simulink model "Wind_Turbine_Flexible_Blades"  (R2025a)
settings: Solver=ode15s  StartTime=0.0  StopTime=10  RelTol=1e-5  EnableMultiTasking=on
PreLoadFcn:
  | load ss_cantilever_pva.mat
  | warning('off','Simulink:SL_SaveWithParameterizedLinks_Warning');
PostLoadFcn:
  | loadMass = 20; %kg
InitFcn:
  | cantilever1=cantilever_aluminum;
  | load1.mass = 20 ; %kg
  | load1.inertia = eye(3) ; % assume point mass
  | load2=load1;
  | load2.angle = 35 * pi / 180;
undefined symbols (not defined in the file or in its folder): Extr_Data_Ellipse, WT_Params, X, Y, Z
libraries: sm_lib x22, nesl_utility x7, Pitch_System_Lib x3, Hub_Axis_Lib x1
Description:
  | Copyright 2009-2025 The MathWorks, Inc. MathWorks, Inc.
settings Model: Creator=smiller  LastModifiedBy=smiller
settings SolverCC: AlgebraicLoopSolver=TrustRegion
settings DataIOCC: LimitDataPoints=on  SaveFormat=Array  SignalLoggingSaveFormat=ModelDataLogs  ReturnWorkspaceOutputs=off
settings OptimizationCC: ReuseModelBlockBuffer=off  ExpressionDepthLimit=2147483647.0  InitFltsAndDblsToZero=on  LifeSpan=inf
settings DebuggingCC: AlgebraicLoopMsg=none  ArtificialAlgebraicLoopMsg=none  UnderspecifiedInitializationDetection=Classic  MergeDetectMultiDrivingBlocksExec=none  FcnCallInpInsideContextMsg=warning  UnconnectedInputMsg=warning  UnconnectedOutputMsg=warning  UnconnectedLineMsg=warning  AllowSymbolicDim=off  StateNameClashWarn=warning  PregeneratedLibrarySubsystemCodeDiagnostic=none  SFUnexpectedBacktrackingDiag=warning  SFNoUnconditionalDefaultTransitionDiag=warning  SFExecutionAtInitializationDiag=none  ArithmeticOperatorsInVariantConditions=warning
settings HardwareCC: ProdBitPerPointer=32.0  ProdBitPerSizeT=32.0  ProdBitPerPtrDiffT=32.0  ProdLargestAtomicFloat=None  ProdIntDivRoundTo=Undefined  ProdEndianess=Unspecified  ProdWordSize=32.0  ProdHWDeviceType=32-bit Generic
settings ModelReferenceCC: EnableRefExpFcnMdlSchedulingChecks=on  PropagateSignalLabelsOutOfModel=off
settings SFSimCC: SimUseLocalCustomCode=off  CustomCodeUndefinedFunction=UseInterfaceOnly
settings RTWCC: RTWUseLocalCustomCode=off  GPUComputeCapability=3.5  DLArmComputeVersion=19.05
settings CodeAppCC: StateflowObjectComments=on
settings GRTTargetCC: TargetLangStandard=C89/C90 (ANSI)  CombineOutputUpdateFcns=off  GRTInterface=on
settings ConfigComp: CovMetricSettings=dw  CovSaveCumulativeToWorkspaceVar=on  CovSaveSingleToWorkspaceVar=on  CovExternalEMLEnable=off  CovSFcnEnable=off
settings SimscapeCC: SimscapeNormalizeSystem=off  SimscapeNominalValues="[{\"value\":\"10\",\"unit\":\"V\"},{\"value\":\"1\",\"unit\":\"A\"},{\"value\":\"10\",\"unit\":\"N*m\"},{\"value\":\"10\",\"unit\":\"bar\"},{\"value\":\"100\",\"unit\":\"kJ/kg\"},{\"value\":\"1\",\"unit\":\"kW\"},{\"value\":\"300\",\"unit\":\"K\"},{\"value\":\"100\",\"unit\":\"cm^3/s\"},{\"value\":\"1\",\"unit\":\"kN\"},{\"value\":\"1\",\"unit\":\"g/cm^3\"},{\"value\":\"1\",\"unit\":\"l\"},{\"value\":\"1\",\"unit\":\"cm^2\"},{\"value\":\"60\",\"unit\":\"Hz\"}]"
settings ConfigurationSet: Description=SimMechanics 2G
settings ExplorerConfigSet: InternalSimMechanicsExplorerSettings="<ExplorerConfiguration><canonicalview>default</canonicalview><AnimationSetting><BasePlaybackSpeed>1.0</BasePlaybackSpeed><PlaybackSpeedFactor>1.0</PlaybackSpeedFactor></AnimationSetting><TilePanel><TileInfo><Tiles Columns=\"1\" Count=\"1\" Rows=\"1\"><Column Weight=\"1\"/><Row Weight=\"1\"/><Tile Height=\"1\" Width=\"1\" X=\"0\" Y=\"0\"/></Tiles></TileInfo><SceneInfo><SceneViewer><BGColor><R>1</R><G>1</G><B>1</B></BGColor><Camera><DoPerspective>off</DoPerspective><Position><X>22.7951904532356409</X><Y>25.5078554918571712</Y><Z>43.6986236453718746</Z></Position><Center><X>-2.12432004859473977</X><Y>6.83325398558179486</Y><Z>-1.8734629381775747</Z></Center><Up><X>-0.455754206605199275</X><Y>0.882954249233147026</Y><Z>-0.112605048389475049</Z></Up><ViewLimDist>1</ViewLimDist><YLim>36.0998057556152361</YLim><XLim>37.6274144624230047</XLim></Camera></SceneViewer></SceneInfo></TilePanel><MechEditorPanel><Cameras/><GfxPanelCameraMap/><VideoCreator><PlaybackSpeedRatio>1.0</PlaybackSpeedRatio><FrameRate>30</FrameRate><VideoFormat>Motion JPEG AVI</VideoFormat><FrameSize>auto</FrameSize></VideoCreator></MechEditorPanel></ExplorerConfiguration>"

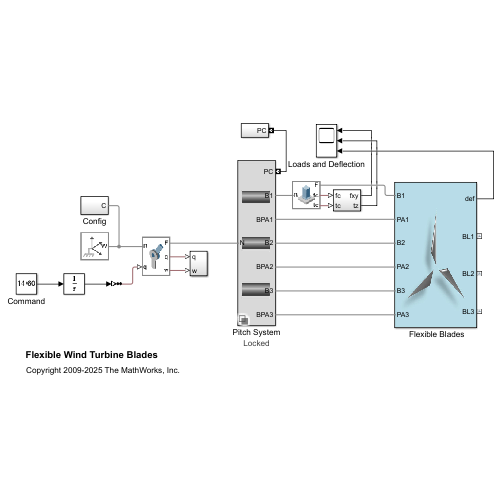
[thumbnail: Simulink's stored preview of the top-level diagram]
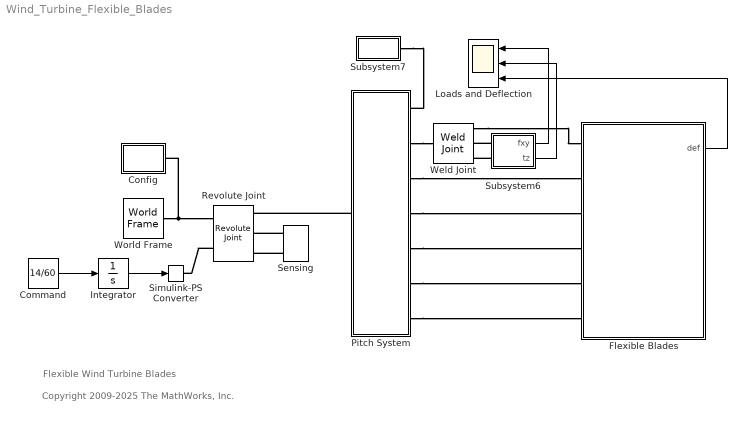
== system Wind_Turbine_Flexible_Blades ==
  note: Copyright 2009-2025 The MathWorks, Inc.
  note: Flexible Wind Turbine Blades
  " Flexible Blades" : Subsystem
      mask Display: image('Blades_IMAGE.jpg');
  Command : Constant  Value=14/60
  Config : Subsystem
  Integrator : Integrator
  Loads and Deflection : Scope  NumInputPorts=3
      settings: ActiveDisplayYMinimum=-4.81536855554E+6  ActiveDisplayYMaximum=1.42317027303E+6  DataLoggingVariableName=ScopeData3
  Pitch System : Subsystem  Tag=CustomStyle  Variant=on  VariantControlMode=label  LabelModeActiveChoice=Locked
      settings: AttributesFormatString=%<ActiveVariant>
      mask Display:
      | blk = wind_turbine_activeVariantBlock(gcb);
      | eval(get_param(blk, 'MaskDisplay'));
  Revolute Joint : sm_lib/Joints/Revolute Joint  JointMode=Normal  CompositeWrenchDir=FollowerOnBase  CompositeWrenchFrame=BaseFrame  SenseConstraintForce=off  SenseConstraintTorque=off  SenseTotalForce=off  SenseTotalTorque=off  PositionTargetSpecify=on  PositionTargetPriority=High  PositionTargetValue=0  PositionTargetValueUnits=deg  VelocityTargetSpecify=off  VelocityTargetPriority=High  VelocityTargetValue=0  VelocityTargetValueUnits=deg/s  EquilibriumPosition=0  EquilibriumPositionUnits=deg  SpringStiffness=0  SpringStiffnessUnits=N*m/deg  DampingCoefficient=0  DampingCoefficientUnits=N*m/(deg/s)  LowerLimitSpecify=off  LowerLimitBound=-90  LowerLimitBoundUnits=deg  LowerLimitStiffness=1e4  LowerLimitStiffnessUnits=N*m/deg  LowerLimitDamping=10  LowerLimitDampingUnits=N*m/(deg/s)  LowerLimitTransitionRegionWidth=0.1  LowerLimitTransitionRegionWidthUnits=deg  UpperLimitSpecify=off  UpperLimitBound=90  UpperLimitBoundUnits=deg  UpperLimitStiffness=1e4  UpperLimitStiffnessUnits=N*m/deg  UpperLimitDamping=10  UpperLimitDampingUnits=N*m/(deg/s)  UpperLimitTransitionRegionWidth=0.1  UpperLimitTransitionRegionWidthUnits=deg  TorqueActuationMode=ComputedTorque  MotionActuationMode=InputMotion  SensePosition=on  SenseVelocity=on  SenseAcceleration=off  SenseTorqueForce=off  SenseLowerLimitTorqueForce=off  SenseUpperLimitTorqueForce=off
  Sensing : Hub_Axis_Lib/Rotate/Sensing  SystemSampleTime=-1  VariantActivationTime=update diagram  EmptyChoice=off  PassThrough=off  PassThroughVariantControl=(default)  EmptyChoiceVariantControl=(default)  AllowFlexibleInterface=on  Latency=0  AutoFrameSizeCalculation=off
  Simulink-PS Converter : nesl_utility/Simulink-PS Converter  PhysicalDomain=network_engine_domain  SubClassName=ps_input  LeftPortType=input  RightPortType=output  PseudoPeriodic=off  Frequencies=[]  NoiseDistribution=none  NoiseParameters=[]  Unit=rev  AffineConversion=off  FilteringAndDerivatives=filter  SimscapeFilterOrder=2  InputFilterTimeConstant=4  UdotUserProvided=0
  Subsystem6 : Subsystem
  Subsystem7 : Subsystem
  Weld Joint : sm_lib/Joints/Weld Joint  JointMode=Normal  CompositeWrenchDir=FollowerOnBase  CompositeWrenchFrame=BaseFrame  SenseConstraintForce=on  SenseConstraintTorque=on  SenseTotalForce=off  SenseTotalTorque=off
  World Frame : sm_lib/Frames and Transforms/World Frame
  wires:
  Command/1 -> Integrator/1
  Subsystem6/1(fxy) -> Loads and Deflection/1
  Subsystem6/2(tz) -> Loads and Deflection/2
  Integrator/1 -> Simulink-PS Converter/1
  " Flexible Blades"/1(def) -> Loads and Deflection/3
  connections:
  Pitch System/LConn6 -- " Flexible Blades"/LConn5
  Pitch System/LConn5 -- " Flexible Blades"/LConn4
  Pitch System/RConn1 -- Revolute Joint/RConn1
  Sensing/LConn1 -- Revolute Joint/RConn2
  Pitch System/LConn2 -- Weld Joint/LConn1
  Pitch System/LConn4 -- " Flexible Blades"/LConn3
  Pitch System/LConn3 -- " Flexible Blades"/LConn2
  Sensing/LConn2 -- Revolute Joint/RConn3
  Pitch System/LConn7 -- " Flexible Blades"/LConn6
  World Frame/RConn1 -- Config/LConn1 -- Revolute Joint/LConn1
  Weld Joint/RConn1 -- " Flexible Blades"/LConn1
  Subsystem6/LConn1 -- Weld Joint/RConn2
  Subsystem6/LConn2 -- Weld Joint/RConn3
  Revolute Joint/LConn2 -- Simulink-PS Converter/RConn1
  Subsystem7/LConn1 -- Pitch System/LConn1

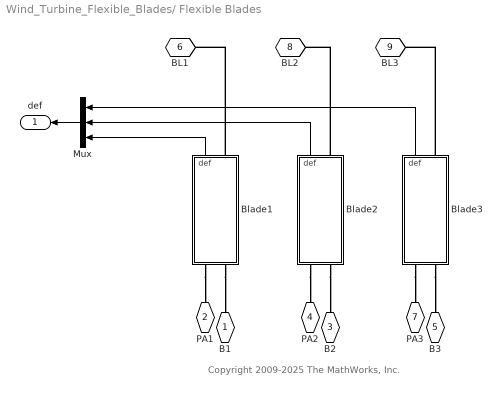
== system Wind_Turbine_Flexible_Blades/ Flexible Blades ==
  note: Copyright 2009-2025 The MathWorks, Inc.
  Blade1 : Subsystem
  Blade2 : Subsystem
  Blade3 : Subsystem
  Mux : Mux  Inputs=3
  B1 : PMIOPort  Tag=PMCPort  Side=Left
  PA1 : PMIOPort  Tag=PMCPort  Port=2  Side=Left
  B2 : PMIOPort  Tag=PMCPort  Port=3  Side=Left
  PA2 : PMIOPort  Tag=PMCPort  Port=4  Side=Left
  B3 : PMIOPort  Tag=PMCPort  Port=5  Side=Left
  BL1 : PMIOPort  Tag=PMCPort  Port=6  Side=Right
  PA3 : PMIOPort  Tag=PMCPort  Port=7  Side=Left
  BL2 : PMIOPort  Tag=PMCPort  Port=8  Side=Right
  BL3 : PMIOPort  Tag=PMCPort  Port=9  Side=Right
  def : Outport  VectorParamsAs1DForOutWhenUnconnected=off
  wires:
  Blade1/1(def) -> Mux/3
  Blade2/1(def) -> Mux/2
  Blade3/1(def) -> Mux/1
  Mux/1 -> def/1
  connections:
  Blade3/LConn1 -- PA3/RConn1
  Blade3/RConn1 -- BL3/RConn1
  Blade3/LConn2 -- B3/RConn1
  Blade2/LConn2 -- B2/RConn1
  Blade2/RConn1 -- BL2/RConn1
  Blade2/LConn1 -- PA2/RConn1
  Blade1/LConn2 -- B1/RConn1
  Blade1/LConn1 -- PA1/RConn1
  Blade1/RConn1 -- BL1/RConn1

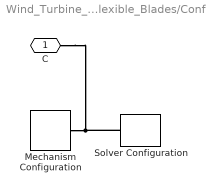
== system Wind_Turbine_Flexible_Blades/Config ==
  Mechanism Configuration : sm_lib/Utilities/Mechanism Configuration  UniformGravity=Constant  GravityVector=[0 0 -9.81]  GravityVectorUnits=m/s^2  LinearizationDelta=0.001  JointModeTransitionNonlinearIterations=2
  Solver Configuration : nesl_utility/Solver Configuration  PhysicalDomain=network_engine_domain  SubClassName=solver  LeftPortType=input  RightPortType=generic  Tones=[]  Harmonics=[]  SimulateNoise=off  Profile=off  UseLocalSampling=off  EnableSwitchedLinearOptims=on  FrequencyDomain=off  UseCCode=off  RelTol=0.001  AbsTol=1e-06  MinStep=1e-09  ToWorkspace=off  RevertToSquareIcSolve=off  NumHomotopyIterations=100  PhasorMode=off  PhasorModeNumHarmonics=1  ConsistencySolver=NEWTON_FTOL  IndexReductionMethod=DerivativeReplacement  DoDC=off  ResidualTolerance=1e-9  ConsistencyTolSource=GLOBAL  ConsistencyAbsTol=0.001  ConsistencyRelTol=0.001  ConsistencyTolFactor=0.001  UseLocalSolver=off  LocalSolverChoice=NE_BACKWARD_EULER_ADVANCER  ResolveIndetEquations=on  FunctionEvalNumThread=1  LocalSolverSampleTime=.001  DoFixedCost=off  MaxNonlinIter=3  MaxModeIter=2  ComputeImpulses=off  ImpulseIterations=2  LinearAlgebra=Sparse  LinearAlgebraNumThread=0  EquationFormulation=NE_TIME_EF  DelaysMemoryBudget=1024  AutomaticFiltering=on  FilteringTimeConstant=0.001  PartitionStorageMethod=AS_NEEDED  PartitionMemoryBudget=1024  PartitionMethod=FAST  MultibodyUseLocalSolver=off  MultibodyLocalSolverChoice=ODE1  MultibodyLocalSolverSampleTime=0.001
  C : PMIOPort  Side=Left
  connections:
  Solver Configuration/RConn1 -- C/RConn1 -- Mechanism Configuration/RConn1

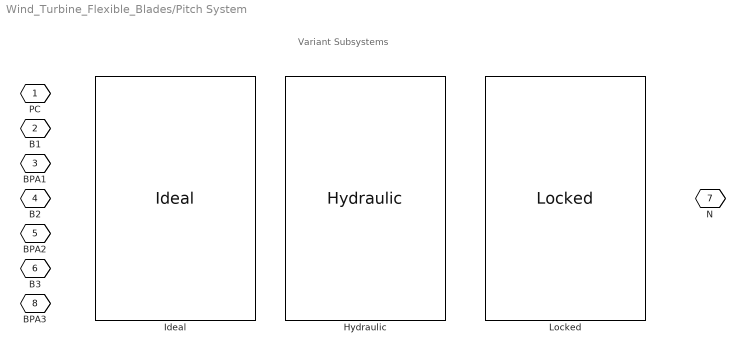
== system Wind_Turbine_Flexible_Blades/Pitch System ==
  note: Variant Subsystems
  Hydraulic : Pitch_System_Lib/Hydraulic  SystemSampleTime=-1  VariantControl=Hydraulic  VariantActivationTime=update diagram  EmptyChoice=off  PassThrough=off  PassThroughVariantControl=(default)  EmptyChoiceVariantControl=(default)  AllowFlexibleInterface=on  Latency=0  AutoFrameSizeCalculation=off
  Ideal : Pitch_System_Lib/Ideal  SystemSampleTime=-1  VariantControl=Ideal  VariantActivationTime=update diagram  EmptyChoice=off  PassThrough=off  PassThroughVariantControl=(default)  EmptyChoiceVariantControl=(default)  AllowFlexibleInterface=on  Latency=0  AutoFrameSizeCalculation=off
  Locked : Pitch_System_Lib/Locked  SystemSampleTime=-1  VariantControl=Locked  VariantActivationTime=update diagram  EmptyChoice=off  PassThrough=off  PassThroughVariantControl=(default)  EmptyChoiceVariantControl=(default)  AllowFlexibleInterface=on  Latency=0  AutoFrameSizeCalculation=off
  PC : PMIOPort  Tag=PMCPort  Side=Left
  B1 : PMIOPort  Tag=PMCPort  Port=2  Side=Left
  BPA1 : PMIOPort  Tag=PMCPort  Port=3  Side=Left
  B2 : PMIOPort  Tag=PMCPort  Port=4  Side=Left
  BPA2 : PMIOPort  Tag=PMCPort  Port=5  Side=Left
  B3 : PMIOPort  Tag=PMCPort  Port=6  Side=Left
  N : PMIOPort  Tag=PMCPort  Port=7  Side=Right
  BPA3 : PMIOPort  Tag=PMCPort  Port=8  Side=Left

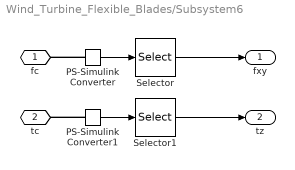
== system Wind_Turbine_Flexible_Blades/Subsystem6 ==
  PS-Simulink Converter : nesl_utility/PS-Simulink Converter  PhysicalDomain=network_engine_domain  SubClassName=ps_output  LeftPortType=input  RightPortType=output  PseudoPeriodic=off  Frequencies=[]  VectorFormat=1-D array  Unit=1  AffineConversion=off
  PS-Simulink Converter1 : nesl_utility/PS-Simulink Converter  PhysicalDomain=network_engine_domain  SubClassName=ps_output  LeftPortType=input  RightPortType=output  PseudoPeriodic=off  Frequencies=[]  VectorFormat=1-D array  Unit=1  AffineConversion=off
  Selector : Selector  InputPortWidth=3  IndexOptions=Index vector (dialog)  Indices=[1 2]  OutputSizes=1
  Selector1 : Selector  InputPortWidth=3  IndexOptions=Index vector (dialog)  Indices=[3]  OutputSizes=1
  fc : PMIOPort  Side=Left
  tc : PMIOPort  Port=2  Side=Left
  fxy : Outport  VectorParamsAs1DForOutWhenUnconnected=off
  tz : Outport  Port=2  VectorParamsAs1DForOutWhenUnconnected=off
  wires:
  PS-Simulink Converter/1 -> Selector/1
  PS-Simulink Converter1/1 -> Selector1/1
  Selector/1 -> fxy/1
  Selector1/1 -> tz/1
  connections:
  PS-Simulink Converter1/LConn1 -- tc/RConn1
  PS-Simulink Converter/LConn1 -- fc/RConn1

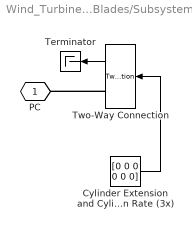
== system Wind_Turbine_Flexible_Blades/Subsystem7 ==
  Cylinder Extension and Cylinder Extension Rate (3x) : Constant  Value=[0 0 0 0 0 0]
  Terminator : Terminator
  Two-Way Connection : TwoWayConnection
  PC : PMIOPort  Tag=PMCPort  Side=Left
  wires:
  Two-Way Connection/1 -> Terminator/1
  Cylinder Extension and Cylinder Extension Rate (3x)/1 -> Two-Way Connection/1
  connections:
  Two-Way Connection/RConn1 -- PC/RConn1

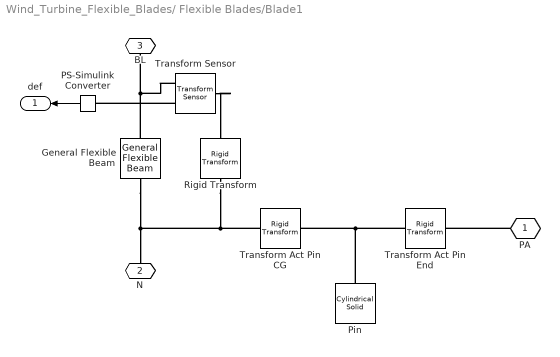
== system Wind_Turbine_Flexible_Blades/ Flexible Blades/Blade1 ==
  General Flexible Beam : sm_lib/Body Elements/Flexible Bodies/Beams/General Flexible Beam  ExtrusionCrossSection=Extr_Data_Ellipse(0.5,1.5,0,359,1)  ExtrusionCrossSectionUnits=m  ExtrusionLength=40  ExtrusionLengthUnits=m  StiffnessAndInertiaType=CalculateFromGeometry  Density=2700  DensityUnits=kg/m^3  ModuliType=YoungsPoissons  YoungsModulus=70  YoungsModulusUnits=GPa  PoissonsRatio=0.33  ShearModulus=26  ShearModulusUnits=GPa  GeometricCentroid=[0 0]  GeometricCentroidUnits=m  BendingCentroid=[0 0]  BendingCentroidUnits=m  ShearCenter=[0 0]  ShearCenterUnits=m  AxialRigidity=1  AxialRigidityUnits=Pa*m^2  FlexuralRigidity=[1 1]  FlexuralRigidityUnits=Pa*m^4  CrossFlexuralRigidity=0  CrossFlexuralRigidityUnits=Pa*m^4  TorsionalRigidity=1  TorsionalRigidityUnits=Pa*m^4  CenterOfMass=[0 0]  CenterOfMassUnits=m  MassPerUnitLength=1  MassPerUnitLengthUnits=kg/m  MassMomentOfInertiaDensity=[1 1]  MassMomentOfInertiaDensityUnits=kg*m  MassProductOfInertiaDensity=0  MassProductOfInertiaDensityUnits=kg*m  DampingType=Proportional  ProportionalDampingAlpha=0  ProportionalDampingAlphaUnits=1/s  ProportionalDampingBeta=0.001  ProportionalDampingBetaUnits=s  UniformModalDampingRatio=0.01  NumElements=1  ReferenceConditionsType=LinearizedMeanAxes  DoExposeReferenceFrame=off  ReductionType=None  NumRetainedModes=1  GraphicType=FromGeometry  GraphicVisPropType=SimpleVisualProperties  GraphicDiffuseColor=[0.5 0.5 0.5]  GraphicOpacity=1.0  GraphicSpecularColor=[0.5 0.5 0.5 1.0]  GraphicAmbientColor=[0.15 0.15 0.15 1.0]  GraphicEmissiveColor=[0.0 0.0 0.0 1.0]  GraphicShininess=75  DoExposeZminFrame=on  DoExposeZmaxFrame=on  SerializedFrames=<Frames/>
  PS-Simulink Converter : nesl_utility/PS-Simulink Converter  PhysicalDomain=network_engine_domain  SubClassName=ps_output  LeftPortType=input  RightPortType=output  PseudoPeriodic=off  Frequencies=[]  VectorFormat=1-D array  Unit=1  AffineConversion=off
  Pin : sm_lib/Body Elements/Cylindrical Solid  CylinderRadius=0.1  CylinderRadiusUnits=m  CylinderLength=-WT_Params.Blade.Actuator_Offset.y  CylinderLengthUnits=m  ExportEntireGeometry=off  InertiaType=PointMass  BasedOnType=Density  Density=1000  DensityUnits=kg/(m^3)  Mass=0.001  MassUnits=kg  CenterOfMass=[0 0 0]  CenterOfMassUnits=m  MomentsOfInertia=[1 1 1]  MomentsOfInertiaUnits=kg*m^2  ProductsOfInertia=[0 0 0]  ProductsOfInertiaUnits=kg*m^2  GraphicType=FromGeometry  MarkerShape=Sphere  MarkerSize=10  GraphicVisPropType=SimpleVisualProperties  GraphicDiffuseColor=[0.6 0.2 0.0]  GraphicOpacity=1.0  GraphicSpecularColor=[0.5 0.5 0.5 1.0]  GraphicAmbientColor=[0.15 0.15 0.15 1.0]  GraphicEmissiveColor=[0.0 0.0 0.0 1.0]  GraphicShininess=75  DoExposeReferenceFrame=on  SerializedFrames=<Frames/>
  Rigid Transform : sm_lib/Frames and Transforms/Rigid Transform  RotationMethod=None  FollAlignAxisA=+X  BaseAlignAxisA=+Y  FollAlignAxisB=+Y  BaseAlignAxisB=+Z  RotationStandardAxis=+Z  RotationAngle=0.0  RotationAngleUnits=deg  RotationArbitraryAxis=[0 0 1]  RotationSequenceAxes=FollowerAxes  RotationSequence=XYX  RotationSequenceAngles=[0 0 0]  RotationSequenceAnglesUnits=deg  RotationMatrix=[1 0 0; 0 1 0; 0 0 1]  Quaternion=[1 0 0 0]  TranslationMethod=StandardAxis  TranslationCartesianOffset=[0 0 0]  TranslationCartesianOffsetUnits=m  TranslationStandardAxis=+Z  TranslationStandardOffset=40  TranslationStandardOffsetUnits=m  TranslationROffset=0  TranslationROffsetUnits=m  TranslationThetaOffset=0  TranslationThetaOffsetUnits=deg  TranslationZOffset=0  TranslationZOffsetUnits=m
  Transform Act Pin CG : sm_lib/Frames and Transforms/Rigid Transform  RotationMethod=None  FollAlignAxisA=+X  BaseAlignAxisA=+Y  FollAlignAxisB=+Y  BaseAlignAxisB=+Z  RotationStandardAxis=+Z  RotationAngle=0  RotationAngleUnits=deg  RotationArbitraryAxis=[0 0 1]  RotationSequenceAxes=FollowerAxes  RotationSequence=XYX  RotationSequenceAngles=[0 0 0]  RotationSequenceAnglesUnits=deg  RotationMatrix=[1 0 0; 0 1 0; 0 0 1]  Quaternion=[1 0 0 0]  TranslationMethod=Cartesian  TranslationCartesianOffset=[0 WT_Params.Blade.Actuator_Offset.z WT_Params.Blade.Actuator_Offset.y/2]  TranslationCartesianOffsetUnits=m  TranslationStandardAxis=+Z  TranslationStandardOffset=0  TranslationStandardOffsetUnits=m  TranslationROffset=0  TranslationROffsetUnits=m  TranslationThetaOffset=0  TranslationThetaOffsetUnits=deg  TranslationZOffset=0  TranslationZOffsetUnits=m
  Transform Act Pin End : sm_lib/Frames and Transforms/Rigid Transform  RotationMethod=None  FollAlignAxisA=+X  BaseAlignAxisA=+Y  FollAlignAxisB=+Y  BaseAlignAxisB=+Z  RotationStandardAxis=+Z  RotationAngle=0  RotationAngleUnits=deg  RotationArbitraryAxis=[0 0 1]  RotationSequenceAxes=FollowerAxes  RotationSequence=XYX  RotationSequenceAngles=[0 0 0]  RotationSequenceAnglesUnits=deg  RotationMatrix=[1 0 0; 0 1 0; 0 0 1]  Quaternion=[1 0 0 0]  TranslationMethod=Cartesian  TranslationCartesianOffset=[0 0 WT_Params.Blade.Actuator_Offset.y/2]  TranslationCartesianOffsetUnits=m  TranslationStandardAxis=+Z  TranslationStandardOffset=0  TranslationStandardOffsetUnits=m  TranslationROffset=0  TranslationROffsetUnits=m  TranslationThetaOffset=0  TranslationThetaOffsetUnits=deg  TranslationZOffset=0  TranslationZOffsetUnits=m
  Transform Sensor : sm_lib/Frames and Transforms/Transform Sensor  MeasurementFrame=World  RotationSequence=XYX  SenseAngle=off  SenseAxis=off  SenseQ=off  SenseR=off  SenseRotationSequence=off  SenseOmegaX=off  SenseOmegaY=off  SenseOmegaZ=off  SenseOmega=off  SenseQDot=off  SenseRDot=off  SenseRotationSequenceDot=off  SenseAlphaX=off  SenseAlphaY=off  SenseAlphaZ=off  SenseAlpha=off  SenseQDDot=off  SenseRDDot=off  SenseX=off  SenseY=off  SenseZ=off  SenseXYZ=off  SenseRad=on  SenseAzim=off  SenseDist=off  SenseInc=off  SenseXDot=off  SenseYDot=off  SenseZDot=off  SenseXYZDot=off  SenseRadDot=off  SenseAzimDot=off  SenseDistDot=off  SenseIncDot=off  SenseXDDot=off  SenseYDDot=off  SenseZDDot=off  SenseXYZDDot=off  SenseRadDDot=off  SenseAzimDDot=off  SenseDistDDot=off  SenseIncDDot=off
  PA : PMIOPort  Side=Left
  N : PMIOPort  Port=2  Side=Left
  BL : PMIOPort  Port=3  Side=Right
  def : Outport  VectorParamsAs1DForOutWhenUnconnected=off
  wires:
  PS-Simulink Converter/1 -> def/1
  connections:
  Pin/RConn1 -- Transform Act Pin End/LConn1 -- Transform Act Pin CG/RConn1
  PA/RConn1 -- Transform Act Pin End/RConn1
  General Flexible Beam/RConn1 -- Transform Sensor/RConn1 -- BL/RConn1
  Transform Act Pin CG/LConn1 -- Rigid Transform/LConn1 -- General Flexible Beam/LConn1 -- N/RConn1
  Transform Sensor/LConn1 -- Rigid Transform/RConn1
  Transform Sensor/RConn2 -- PS-Simulink Converter/LConn1

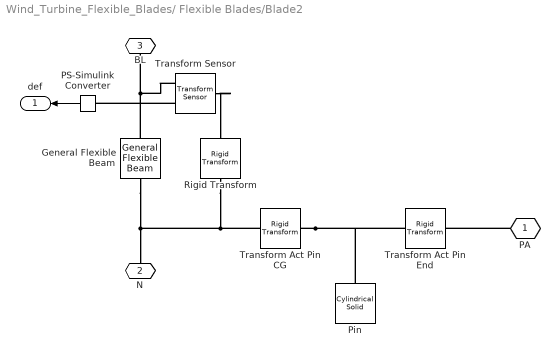
== system Wind_Turbine_Flexible_Blades/ Flexible Blades/Blade2 ==
  General Flexible Beam : sm_lib/Body Elements/Flexible Bodies/Beams/General Flexible Beam  ExtrusionCrossSection=Extr_Data_Ellipse(0.5,1.5,0,359,1)  ExtrusionCrossSectionUnits=m  ExtrusionLength=40  ExtrusionLengthUnits=m  StiffnessAndInertiaType=CalculateFromGeometry  Density=2700  DensityUnits=kg/m^3  ModuliType=YoungsPoissons  YoungsModulus=70  YoungsModulusUnits=GPa  PoissonsRatio=0.33  ShearModulus=26  ShearModulusUnits=GPa  GeometricCentroid=[0 0]  GeometricCentroidUnits=m  BendingCentroid=[0 0]  BendingCentroidUnits=m  ShearCenter=[0 0]  ShearCenterUnits=m  AxialRigidity=1  AxialRigidityUnits=Pa*m^2  FlexuralRigidity=[1 1]  FlexuralRigidityUnits=Pa*m^4  CrossFlexuralRigidity=0  CrossFlexuralRigidityUnits=Pa*m^4  TorsionalRigidity=1  TorsionalRigidityUnits=Pa*m^4  CenterOfMass=[0 0]  CenterOfMassUnits=m  MassPerUnitLength=1  MassPerUnitLengthUnits=kg/m  MassMomentOfInertiaDensity=[1 1]  MassMomentOfInertiaDensityUnits=kg*m  MassProductOfInertiaDensity=0  MassProductOfInertiaDensityUnits=kg*m  DampingType=Proportional  ProportionalDampingAlpha=0  ProportionalDampingAlphaUnits=1/s  ProportionalDampingBeta=0.001  ProportionalDampingBetaUnits=s  UniformModalDampingRatio=0.01  NumElements=1  ReferenceConditionsType=LinearizedMeanAxes  DoExposeReferenceFrame=off  ReductionType=None  NumRetainedModes=1  GraphicType=FromGeometry  GraphicVisPropType=SimpleVisualProperties  GraphicDiffuseColor=[0.5 0.5 0.5]  GraphicOpacity=1.0  GraphicSpecularColor=[0.5 0.5 0.5 1.0]  GraphicAmbientColor=[0.15 0.15 0.15 1.0]  GraphicEmissiveColor=[0.0 0.0 0.0 1.0]  GraphicShininess=75  DoExposeZminFrame=on  DoExposeZmaxFrame=on  SerializedFrames=<Frames/>
  PS-Simulink Converter : nesl_utility/PS-Simulink Converter  PhysicalDomain=network_engine_domain  SubClassName=ps_output  LeftPortType=input  RightPortType=output  PseudoPeriodic=off  Frequencies=[]  VectorFormat=1-D array  Unit=1  AffineConversion=off
  Pin : sm_lib/Body Elements/Cylindrical Solid  CylinderRadius=0.1  CylinderRadiusUnits=m  CylinderLength=-WT_Params.Blade.Actuator_Offset.y  CylinderLengthUnits=m  ExportEntireGeometry=off  InertiaType=PointMass  BasedOnType=Density  Density=1000  DensityUnits=kg/(m^3)  Mass=0.001  MassUnits=kg  CenterOfMass=[0 0 0]  CenterOfMassUnits=m  MomentsOfInertia=[1 1 1]  MomentsOfInertiaUnits=kg*m^2  ProductsOfInertia=[0 0 0]  ProductsOfInertiaUnits=kg*m^2  GraphicType=FromGeometry  MarkerShape=Sphere  MarkerSize=10  GraphicVisPropType=SimpleVisualProperties  GraphicDiffuseColor=[0.6 0.2 0.0]  GraphicOpacity=1.0  GraphicSpecularColor=[0.5 0.5 0.5 1.0]  GraphicAmbientColor=[0.15 0.15 0.15 1.0]  GraphicEmissiveColor=[0.0 0.0 0.0 1.0]  GraphicShininess=75  DoExposeReferenceFrame=on  SerializedFrames=<Frames/>
  Rigid Transform : sm_lib/Frames and Transforms/Rigid Transform  RotationMethod=None  FollAlignAxisA=+X  BaseAlignAxisA=+Y  FollAlignAxisB=+Y  BaseAlignAxisB=+Z  RotationStandardAxis=+Z  RotationAngle=0.0  RotationAngleUnits=deg  RotationArbitraryAxis=[0 0 1]  RotationSequenceAxes=FollowerAxes  RotationSequence=XYX  RotationSequenceAngles=[0 0 0]  RotationSequenceAnglesUnits=deg  RotationMatrix=[1 0 0; 0 1 0; 0 0 1]  Quaternion=[1 0 0 0]  TranslationMethod=StandardAxis  TranslationCartesianOffset=[0 0 0]  TranslationCartesianOffsetUnits=m  TranslationStandardAxis=+Z  TranslationStandardOffset=40  TranslationStandardOffsetUnits=m  TranslationROffset=0  TranslationROffsetUnits=m  TranslationThetaOffset=0  TranslationThetaOffsetUnits=deg  TranslationZOffset=0  TranslationZOffsetUnits=m
  Transform Act Pin CG : sm_lib/Frames and Transforms/Rigid Transform  RotationMethod=None  FollAlignAxisA=+X  BaseAlignAxisA=+Y  FollAlignAxisB=+Y  BaseAlignAxisB=+Z  RotationStandardAxis=+Z  RotationAngle=0  RotationAngleUnits=deg  RotationArbitraryAxis=[0 0 1]  RotationSequenceAxes=FollowerAxes  RotationSequence=XYX  RotationSequenceAngles=[0 0 0]  RotationSequenceAnglesUnits=deg  RotationMatrix=[1 0 0; 0 1 0; 0 0 1]  Quaternion=[1 0 0 0]  TranslationMethod=Cartesian  TranslationCartesianOffset=[0 WT_Params.Blade.Actuator_Offset.z WT_Params.Blade.Actuator_Offset.y/2]  TranslationCartesianOffsetUnits=m  TranslationStandardAxis=+Z  TranslationStandardOffset=0  TranslationStandardOffsetUnits=m  TranslationROffset=0  TranslationROffsetUnits=m  TranslationThetaOffset=0  TranslationThetaOffsetUnits=deg  TranslationZOffset=0  TranslationZOffsetUnits=m
  Transform Act Pin End : sm_lib/Frames and Transforms/Rigid Transform  RotationMethod=None  FollAlignAxisA=+X  BaseAlignAxisA=+Y  FollAlignAxisB=+Y  BaseAlignAxisB=+Z  RotationStandardAxis=+Z  RotationAngle=0  RotationAngleUnits=deg  RotationArbitraryAxis=[0 0 1]  RotationSequenceAxes=FollowerAxes  RotationSequence=XYX  RotationSequenceAngles=[0 0 0]  RotationSequenceAnglesUnits=deg  RotationMatrix=[1 0 0; 0 1 0; 0 0 1]  Quaternion=[1 0 0 0]  TranslationMethod=Cartesian  TranslationCartesianOffset=[0 0 WT_Params.Blade.Actuator_Offset.y/2]  TranslationCartesianOffsetUnits=m  TranslationStandardAxis=+Z  TranslationStandardOffset=0  TranslationStandardOffsetUnits=m  TranslationROffset=0  TranslationROffsetUnits=m  TranslationThetaOffset=0  TranslationThetaOffsetUnits=deg  TranslationZOffset=0  TranslationZOffsetUnits=m
  Transform Sensor : sm_lib/Frames and Transforms/Transform Sensor  MeasurementFrame=World  RotationSequence=XYX  SenseAngle=off  SenseAxis=off  SenseQ=off  SenseR=off  SenseRotationSequence=off  SenseOmegaX=off  SenseOmegaY=off  SenseOmegaZ=off  SenseOmega=off  SenseQDot=off  SenseRDot=off  SenseRotationSequenceDot=off  SenseAlphaX=off  SenseAlphaY=off  SenseAlphaZ=off  SenseAlpha=off  SenseQDDot=off  SenseRDDot=off  SenseX=off  SenseY=off  SenseZ=off  SenseXYZ=off  SenseRad=on  SenseAzim=off  SenseDist=off  SenseInc=off  SenseXDot=off  SenseYDot=off  SenseZDot=off  SenseXYZDot=off  SenseRadDot=off  SenseAzimDot=off  SenseDistDot=off  SenseIncDot=off  SenseXDDot=off  SenseYDDot=off  SenseZDDot=off  SenseXYZDDot=off  SenseRadDDot=off  SenseAzimDDot=off  SenseDistDDot=off  SenseIncDDot=off
  PA : PMIOPort  Side=Left
  N : PMIOPort  Port=2  Side=Left
  BL : PMIOPort  Port=3  Side=Right
  def : Outport  VectorParamsAs1DForOutWhenUnconnected=off
  wires:
  PS-Simulink Converter/1 -> def/1
  connections:
  Transform Sensor/RConn2 -- PS-Simulink Converter/LConn1
  Transform Sensor/LConn1 -- Rigid Transform/RConn1
  Rigid Transform/LConn1 -- Transform Act Pin CG/LConn1 -- N/RConn1 -- General Flexible Beam/LConn1
  Transform Sensor/RConn1 -- General Flexible Beam/RConn1 -- BL/RConn1
  PA/RConn1 -- Transform Act Pin End/RConn1
  Transform Act Pin CG/RConn1 -- Transform Act Pin End/LConn1 -- Pin/RConn1

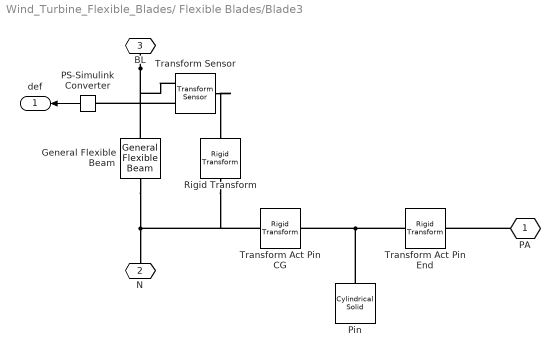
== system Wind_Turbine_Flexible_Blades/ Flexible Blades/Blade3 ==
  General Flexible Beam : sm_lib/Body Elements/Flexible Bodies/Beams/General Flexible Beam  ExtrusionCrossSection=Extr_Data_Ellipse(0.5,1.5,0,359,1)  ExtrusionCrossSectionUnits=m  ExtrusionLength=40  ExtrusionLengthUnits=m  StiffnessAndInertiaType=CalculateFromGeometry  Density=2700  DensityUnits=kg/m^3  ModuliType=YoungsPoissons  YoungsModulus=70  YoungsModulusUnits=GPa  PoissonsRatio=0.33  ShearModulus=26  ShearModulusUnits=GPa  GeometricCentroid=[0 0]  GeometricCentroidUnits=m  BendingCentroid=[0 0]  BendingCentroidUnits=m  ShearCenter=[0 0]  ShearCenterUnits=m  AxialRigidity=1  AxialRigidityUnits=Pa*m^2  FlexuralRigidity=[1 1]  FlexuralRigidityUnits=Pa*m^4  CrossFlexuralRigidity=0  CrossFlexuralRigidityUnits=Pa*m^4  TorsionalRigidity=1  TorsionalRigidityUnits=Pa*m^4  CenterOfMass=[0 0]  CenterOfMassUnits=m  MassPerUnitLength=1  MassPerUnitLengthUnits=kg/m  MassMomentOfInertiaDensity=[1 1]  MassMomentOfInertiaDensityUnits=kg*m  MassProductOfInertiaDensity=0  MassProductOfInertiaDensityUnits=kg*m  DampingType=Proportional  ProportionalDampingAlpha=0  ProportionalDampingAlphaUnits=1/s  ProportionalDampingBeta=0.001  ProportionalDampingBetaUnits=s  UniformModalDampingRatio=0.01  NumElements=1  ReferenceConditionsType=LinearizedMeanAxes  DoExposeReferenceFrame=off  ReductionType=None  NumRetainedModes=1  GraphicType=FromGeometry  GraphicVisPropType=SimpleVisualProperties  GraphicDiffuseColor=[0.5 0.5 0.5]  GraphicOpacity=1.0  GraphicSpecularColor=[0.5 0.5 0.5 1.0]  GraphicAmbientColor=[0.15 0.15 0.15 1.0]  GraphicEmissiveColor=[0.0 0.0 0.0 1.0]  GraphicShininess=75  DoExposeZminFrame=on  DoExposeZmaxFrame=on  SerializedFrames=<Frames/>
  PS-Simulink Converter : nesl_utility/PS-Simulink Converter  PhysicalDomain=network_engine_domain  SubClassName=ps_output  LeftPortType=input  RightPortType=output  PseudoPeriodic=off  Frequencies=[]  VectorFormat=1-D array  Unit=1  AffineConversion=off
  Pin : sm_lib/Body Elements/Cylindrical Solid  CylinderRadius=0.1  CylinderRadiusUnits=m  CylinderLength=-WT_Params.Blade.Actuator_Offset.y  CylinderLengthUnits=m  ExportEntireGeometry=off  InertiaType=PointMass  BasedOnType=Density  Density=1000  DensityUnits=kg/(m^3)  Mass=0.001  MassUnits=kg  CenterOfMass=[0 0 0]  CenterOfMassUnits=m  MomentsOfInertia=[1 1 1]  MomentsOfInertiaUnits=kg*m^2  ProductsOfInertia=[0 0 0]  ProductsOfInertiaUnits=kg*m^2  GraphicType=FromGeometry  MarkerShape=Sphere  MarkerSize=10  GraphicVisPropType=SimpleVisualProperties  GraphicDiffuseColor=[0.6 0.2 0.0]  GraphicOpacity=1.0  GraphicSpecularColor=[0.5 0.5 0.5 1.0]  GraphicAmbientColor=[0.15 0.15 0.15 1.0]  GraphicEmissiveColor=[0.0 0.0 0.0 1.0]  GraphicShininess=75  DoExposeReferenceFrame=on  SerializedFrames=<Frames/>
  Rigid Transform : sm_lib/Frames and Transforms/Rigid Transform  RotationMethod=None  FollAlignAxisA=+X  BaseAlignAxisA=+Y  FollAlignAxisB=+Y  BaseAlignAxisB=+Z  RotationStandardAxis=+Z  RotationAngle=0.0  RotationAngleUnits=deg  RotationArbitraryAxis=[0 0 1]  RotationSequenceAxes=FollowerAxes  RotationSequence=XYX  RotationSequenceAngles=[0 0 0]  RotationSequenceAnglesUnits=deg  RotationMatrix=[1 0 0; 0 1 0; 0 0 1]  Quaternion=[1 0 0 0]  TranslationMethod=StandardAxis  TranslationCartesianOffset=[0 0 0]  TranslationCartesianOffsetUnits=m  TranslationStandardAxis=+Z  TranslationStandardOffset=40  TranslationStandardOffsetUnits=m  TranslationROffset=0  TranslationROffsetUnits=m  TranslationThetaOffset=0  TranslationThetaOffsetUnits=deg  TranslationZOffset=0  TranslationZOffsetUnits=m
  Transform Act Pin CG : sm_lib/Frames and Transforms/Rigid Transform  RotationMethod=None  FollAlignAxisA=+X  BaseAlignAxisA=+Y  FollAlignAxisB=+Y  BaseAlignAxisB=+Z  RotationStandardAxis=+Z  RotationAngle=0  RotationAngleUnits=deg  RotationArbitraryAxis=[0 0 1]  RotationSequenceAxes=FollowerAxes  RotationSequence=XYX  RotationSequenceAngles=[0 0 0]  RotationSequenceAnglesUnits=deg  RotationMatrix=[1 0 0; 0 1 0; 0 0 1]  Quaternion=[1 0 0 0]  TranslationMethod=Cartesian  TranslationCartesianOffset=[0 WT_Params.Blade.Actuator_Offset.z WT_Params.Blade.Actuator_Offset.y/2]  TranslationCartesianOffsetUnits=m  TranslationStandardAxis=+Z  TranslationStandardOffset=0  TranslationStandardOffsetUnits=m  TranslationROffset=0  TranslationROffsetUnits=m  TranslationThetaOffset=0  TranslationThetaOffsetUnits=deg  TranslationZOffset=0  TranslationZOffsetUnits=m
  Transform Act Pin End : sm_lib/Frames and Transforms/Rigid Transform  RotationMethod=None  FollAlignAxisA=+X  BaseAlignAxisA=+Y  FollAlignAxisB=+Y  BaseAlignAxisB=+Z  RotationStandardAxis=+Z  RotationAngle=0  RotationAngleUnits=deg  RotationArbitraryAxis=[0 0 1]  RotationSequenceAxes=FollowerAxes  RotationSequence=XYX  RotationSequenceAngles=[0 0 0]  RotationSequenceAnglesUnits=deg  RotationMatrix=[1 0 0; 0 1 0; 0 0 1]  Quaternion=[1 0 0 0]  TranslationMethod=Cartesian  TranslationCartesianOffset=[0 0 WT_Params.Blade.Actuator_Offset.y/2]  TranslationCartesianOffsetUnits=m  TranslationStandardAxis=+Z  TranslationStandardOffset=0  TranslationStandardOffsetUnits=m  TranslationROffset=0  TranslationROffsetUnits=m  TranslationThetaOffset=0  TranslationThetaOffsetUnits=deg  TranslationZOffset=0  TranslationZOffsetUnits=m
  Transform Sensor : sm_lib/Frames and Transforms/Transform Sensor  MeasurementFrame=World  RotationSequence=XYX  SenseAngle=off  SenseAxis=off  SenseQ=off  SenseR=off  SenseRotationSequence=off  SenseOmegaX=off  SenseOmegaY=off  SenseOmegaZ=off  SenseOmega=off  SenseQDot=off  SenseRDot=off  SenseRotationSequenceDot=off  SenseAlphaX=off  SenseAlphaY=off  SenseAlphaZ=off  SenseAlpha=off  SenseQDDot=off  SenseRDDot=off  SenseX=off  SenseY=off  SenseZ=off  SenseXYZ=off  SenseRad=on  SenseAzim=off  SenseDist=off  SenseInc=off  SenseXDot=off  SenseYDot=off  SenseZDot=off  SenseXYZDot=off  SenseRadDot=off  SenseAzimDot=off  SenseDistDot=off  SenseIncDot=off  SenseXDDot=off  SenseYDDot=off  SenseZDDot=off  SenseXYZDDot=off  SenseRadDDot=off  SenseAzimDDot=off  SenseDistDDot=off  SenseIncDDot=off
  PA : PMIOPort  Side=Left
  N : PMIOPort  Port=2  Side=Left
  BL : PMIOPort  Port=3  Side=Right
  def : Outport  VectorParamsAs1DForOutWhenUnconnected=off
  wires:
  PS-Simulink Converter/1 -> def/1
  connections:
  Pin/RConn1 -- Transform Act Pin End/LConn1 -- Transform Act Pin CG/RConn1
  PA/RConn1 -- Transform Act Pin End/RConn1
  BL/RConn1 -- General Flexible Beam/RConn1 -- Transform Sensor/RConn1
  General Flexible Beam/LConn1 -- N/RConn1 -- Transform Act Pin CG/LConn1 -- Rigid Transform/LConn1
  Transform Sensor/LConn1 -- Rigid Transform/RConn1
  Transform Sensor/RConn2 -- PS-Simulink Converter/LConn1
